simulink model "LQG_nonlinear_sim"  (R2026a)
settings: Solver=ode23t  StopTime=4  MaxStep=0.0050000000000000001  RelTol=1.0000000000000001e-05  AbsTol=9.9999999999999995e-08
InitFcn:
  | actuator = actuator_params_nominal();
  | [Gact, info] = build_nominal_actuator(actuator);
  | 
  | % Parametri del robot
  | p = sea_params_nominal();
  | Simulink.Bus.createObject(p);
  | 
  | % Equilibrio desiderato
  | qbar = [pi/2; 0];
  | 
  | % Calcolo stato e coppia di equilibrio
  | [xbar, taubar, info] = sea_static_equilibrium(qbar, p);
undefined symbols (not defined in the file): A, B, C, K, L, Nr, taubar, xbar
libraries: cstblocks_lti x2
Description:
  | explicit LQR plus Kalman observer -> M3 actuators -> nonlinear M1 SEA
settings Model: Creator=aless  LastModifiedBy=rebec

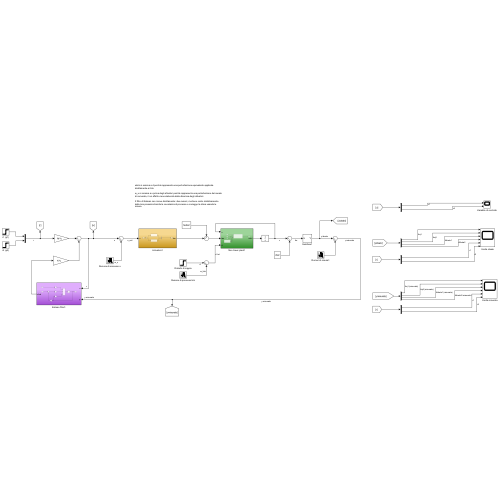
[thumbnail: Simulink's stored preview of the top-level diagram]
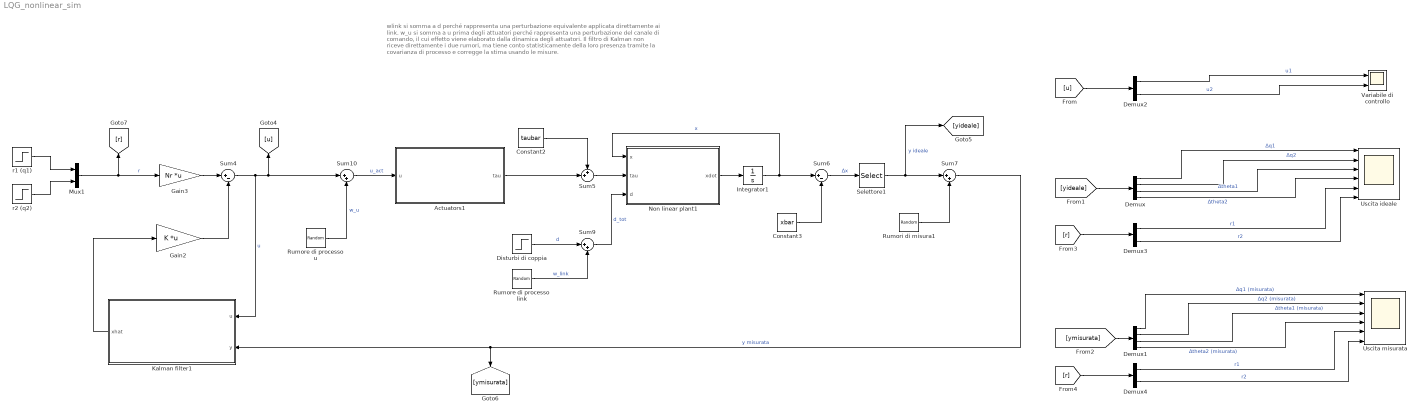
== system LQG_nonlinear_sim ==
  note: wlink​ si somma a d perché rappresenta una perturbazione equivalente applicata direttamente ai link.
      | w_u​ si somma a u prima degli attuatori perché rappresenta una perturbazione del canale di comando, il cui effetto viene elaborato dalla dinamica degli attuatori.
      | Il filtro di Kalman non riceve direttamente i due rumori, ma tiene conto statisticamente della loro presenza tramite la covarianza di processo e corregge la stima usando le misure.
  Actuators1 : Subsystem
  Constant2 : Constant  Value=taubar
  Constant3 : Constant  Value=xbar
  Demux : Demux
  Demux1 : Demux
  Demux2 : Demux  Outputs=2
  Demux3 : Demux  Outputs=2
  Demux4 : Demux  Outputs=2
  Disturbi di coppia : Step  Time=[1 1]  InitialValue=[0 0]  FinalValue=[0.5 0]  SampleTime=0
  Gain2 : Gain  Gain=K  Multiplication=Matrix(K*u)
  Gain3 : Gain  Gain=Nr  Multiplication=Matrix(K*u)
  Integrator1 : Integrator  InitialCondition=xbar
  Kalman filter1 : Subsystem
  Mux1 : Mux  Inputs=2
  Non linear plant1 : Subsystem
  Rumore di processo link : RandomNumber  Mean=[0 0]  Variance=[0.01 0.01]  Seed=20260826  SampleTime=0.002
  Rumore di processo u : RandomNumber  Mean=[0 0]  Variance=[0.01 0.01]  Seed=20260826  SampleTime=0.002
  Rumori di misura1 : RandomNumber  Mean=[0 0 0 0]  Variance=[(0.05*pi/180)^2 (0.05*pi/180)^2 (0.05*pi/180)^2 (0.05*pi/180)^2]  Seed=20260826  SampleTime=0.002
  Selettore1 : Selector  InputPortWidth=8  IndexOptions=Index vector (dialog)  Indices=[1 2 5 6]  OutputSizes=1
  Sum10 : Sum  Inputs=|++
  Sum4 : Sum  Inputs=|+-
  Sum5 : Sum  Inputs=++|
  Sum6 : Sum  Inputs=|+-
  Sum7 : Sum  Inputs=|++
  Sum9 : Sum  Inputs=|++
  Uscita ideale : Scope  NumInputPorts=6
      settings: Title=y (uscita ideale)  ActiveDisplayYMinimum=-0.088271118920575181  ActiveDisplayYMaximum=0.23303114019935003
  Uscita misurata : Scope  NumInputPorts=6
      settings: Title=y (uscita ideale)  ActiveDisplayYMinimum=-0.11442029066688837  ActiveDisplayYMaximum=0.16914890182413583
  Variabile di controllo : Scope  NumInputPorts=2
      settings: ActiveDisplayYMinimum=-2.6959450601265313  ActiveDisplayYMaximum=5.9059369724787079  DataLoggingVariableName=ScopeData2
  r1 (q1) : Step  FinalValue=5*pi/180  SampleTime=0
  r2 (q2) : Step  FinalValue=0  SampleTime=0
  wires:
  Demux/1 -> Uscita ideale/1  "Δq1"
  Demux/2 -> Uscita ideale/2  "Δq2"
  Demux/3 -> Uscita ideale/3  "Δtheta1"
  Demux/4 -> Uscita ideale/4  "Δtheta2"
  Demux1/2 -> Uscita misurata/2  "Δq2 (misurata)"
  Demux1/4 -> Uscita misurata/4  "Δtheta2 (misurata)"
  Demux1/1 -> Uscita misurata/1  "Δq1 (misurata)"
  Demux1/3 -> Uscita misurata/3  "Δtheta1 (misurata)"
  Demux2/1 -> Variabile di controllo/1  "u1"
  Demux2/2 -> Variabile di controllo/2  "u2"
  [u] -> Demux2/1
  [yideale] -> Demux/1
  [ymisurata] -> Demux1/1
  [r] -> Demux3/1
  [r] -> Demux4/1
  Demux3/1 -> Uscita ideale/5  "r1"
  Demux3/2 -> Uscita ideale/6  "r2"
  Demux4/1 -> Uscita misurata/5  "r1"
  Demux4/2 -> Uscita misurata/6  "r2"
  Rumore di processo link/1 -> Sum9/2  "w_link"
  Constant3/1 -> Sum6/2
  Integrator1/1 -> Non linear plant1/1(x), Sum6/1  "x"
  r1 (q1)/1 -> Mux1/1
  Sum7/1 -> [ymisurata], Kalman filter1/2(y)  "y misurata"
  Sum10/1 -> Actuators1/1(u)  "u_act"
  Actuators1/1(tau) -> Sum5/2
  Selettore1/1 -> Sum7/1, [yideale]  "y ideale"
  Gain2/1 -> Sum4/2
  Kalman filter1/1(xhat) -> Gain2/1
  Sum5/1 -> Non linear plant1/2(tau)
  Sum9/1 -> Non linear plant1/3(d)  "d_tot"
  r2 (q2)/1 -> Mux1/2
  Non linear plant1/1(xdot) -> Integrator1/1
  Sum6/1 -> Selettore1/1  "Δx"
  Mux1/1 -> Gain3/1, [r]  "r"
  Disturbi di coppia/1 -> Sum9/1  "d"
  Constant2/1 -> Sum5/1
  Gain3/1 -> Sum4/1
  Rumori di misura1/1 -> Sum7/2
  Sum4/1 -> Kalman filter1/1(u), [u], Sum10/1  "u"
  Rumore di processo u/1 -> Sum10/2  "w_u"

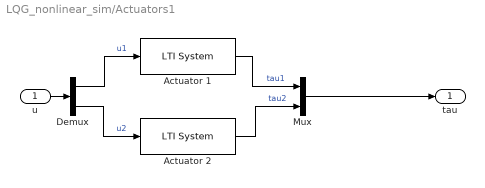
== system LQG_nonlinear_sim/Actuators1 ==
  u : Inport
  Actuator 1 : cstblocks_lti/LTI System  sys=Gact  IC=[]  PadeOrder=0
      settings: LibrarySourceBlock=cstblocks/LTI System
  Actuator 2 : cstblocks_lti/LTI System  sys=Gact  IC=[]  PadeOrder=0
      settings: LibrarySourceBlock=cstblocks/LTI System
  Demux : Demux  Outputs=2
  Mux : Mux  Inputs=2
  tau : Outport
  wires:
  Actuator 2/1 -> Mux/2  "tau2"
  Demux/2 -> Actuator 2/1  "u2"
  u/1 -> Demux/1
  Demux/1 -> Actuator 1/1  "u1"
  Mux/1 -> tau/1
  Actuator 1/1 -> Mux/1  "tau1"

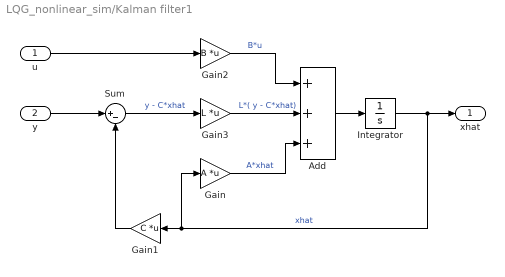
== system LQG_nonlinear_sim/Kalman filter1 ==
  u : Inport
  y : Inport  Port=2
  Add : Sum  Inputs=+++
  Gain : Gain  Gain=A  Multiplication=Matrix(K*u)
  Gain1 : Gain  Gain=C  Multiplication=Matrix(K*u)
  Gain2 : Gain  Gain=B  Multiplication=Matrix(K*u)
  Gain3 : Gain  Gain=L  Multiplication=Matrix(K*u)
  Integrator : Integrator
  Sum : Sum  Inputs=|+-
  xhat : Outport
  wires:
  u/1 -> Gain2/1
  y/1 -> Sum/1
  Gain1/1 -> Sum/2
  Sum/1 -> Gain3/1  "y - C*xhat"
  Gain3/1 -> Add/2  "L*( y - C*xhat)"
  Gain2/1 -> Add/1  "B*u"
  Gain/1 -> Add/3  "A*xhat"
  Add/1 -> Integrator/1
  Integrator/1 -> Gain/1, Gain1/1, xhat/1  "xhat"

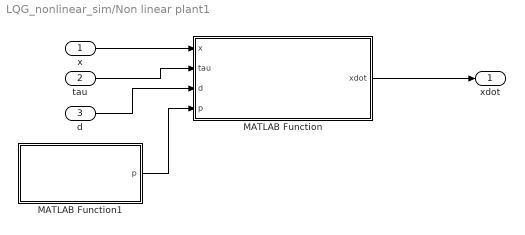
== system LQG_nonlinear_sim/Non linear plant1 ==
  x : Inport
  tau : Inport  Port=2
  d : Inport  Port=3
  MATLAB Function : MATLAB Function  TreatAsAtomicUnit=on
  MATLAB Function1 : MATLAB Function  TreatAsAtomicUnit=on
  xdot : Outport
  wires:
  x/1 -> MATLAB Function/1(x)
  tau/1 -> MATLAB Function/2(tau)
  MATLAB Function/1(xdot) -> xdot/1
  MATLAB Function1/1(p) -> MATLAB Function/4(p)
  d/1 -> MATLAB Function/3(d)

== matlab function LQG_nonlinear_sim/Non linear plant1/MATLAB Function ==
  data: x input; xdot output; tau input; d input; p input
function xdot = sea_nonlinear_rhs_with_link_disturbance(x, tau, d, p)
%SEA_NONLINEAR_RHS_WITH_LINK_DISTURBANCE SEA dynamics with link torque D.
%   TAU remains the motor-side input; D is an external link-side joint
%   torque entering with positive sign in the link equation.

assert(numel(x) == 8, ...
    'sea_nonlinear_rhs_with_link_disturbance:InvalidState', ...
    'The state must contain exactly eight elements.');
assert(numel(tau) == 2 && numel(d) == 2, ...
    'sea_nonlinear_rhs_with_link_disturbance:InvalidInput', ...
    'Both tau and d must contain exactly two elements.');
x = reshape(x, 8, 1);
tau = reshape(tau, 2, 1);
d = reshape(d, 2, 1);

q = x(1:2);
qdot = x(3:4);
theta = x(5:6);
thetadot = x(7:8);
M = sea_link_inertia(q, p);
C = sea_coriolis(q, qdot, p);
G = sea_gravity(q, p);
tauElastic = sea_elastic_torque(q, theta, p);

qddot = M \ (tauElastic + d - C * qdot - G);
thetaddot = p.Jm \ (tau - p.Bm * thetadot - tauElastic);
xdot = [qdot; qddot; thetadot; thetaddot];
end

== matlab function LQG_nonlinear_sim/Non linear plant1/MATLAB Function1 ==
  data: p output Bus: slBus1
function p = sea_params_nominal
%SEA_PARAMS_NOMINAL Nominal mechanical parameters of the 2R SEA robot.
%   P = SEA_PARAMS_NOMINAL returns the values stated by the official
%   assignment. Matrices follow the joint order [joint 1; joint 2].

p.m1 = 1.0;                   % kg
p.m2 = 0.8;                   % kg
p.l1 = 0.4;                   % m
p.l2 = 0.3;                   % m
p.Jm = diag([0.01, 0.01]);    % kg*m^2
p.Bm = diag([0.02, 0.02]);    % N*m*s/rad
p.Ks = diag([50, 40]);        % N*m/rad
p.g = 9.81;                   % m/s^2
end
